simulink model "sfInternalTransitionError"  (R2025b)
settings: Solver=VariableStepAuto  StartTime=0.0  StopTime=10.0  RelTol=1e-3
settings Model: Creator=The MathWorks, Inc.  LastModifiedBy=The MathWorks, Inc.

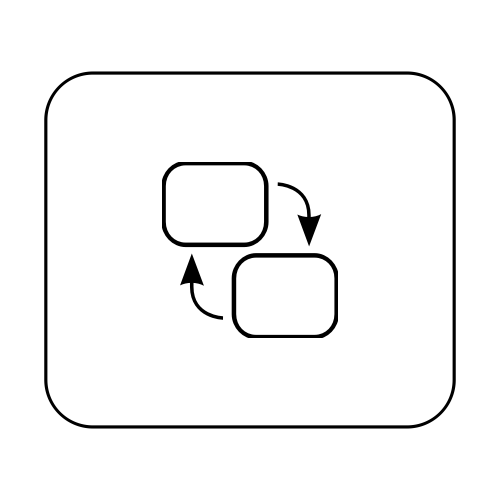
[thumbnail: Simulink's stored preview of the top-level diagram]
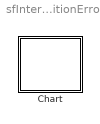
== system sfInternalTransitionError ==
  Chart : Stateflow chart  TreatAsAtomicUnit=on

== stateflow chart sfInternalTransitionError/Chart ==
  state A
    A -> (junction 5) [order 1] : every(1,tick){x=x+1; local}
  (default) -> A
  A -> (junction 15) [order 1] : every(1,tick)
  (junction 16) -> A : {x=x+3;}
  (junction 15) -> (junction 16)
  data: x local =0
  events: local local FUNCTION_CALL_EVENT
